simulink model "Final_year_project_mechanical_fault"  (R2024b)
settings: Solver=ode45  StartTime=0.0  StopTime=20  MaxStep=1e-4  RelTol=1e-3  EnableMultiTasking=on
libraries: spsACVoltageSourceLib x1, spsCurrentMeasurementLib x1, spsRMSLib x1, spsSinglePhaseAsynchronousMachineLib x1, spsVoltageMeasurementLib x1, spspowerguiLib x1
settings Model: Creator=Misty Porcupine  LastModifiedBy=Misty Porcupine
settings SolverCC: AlgebraicLoopSolver=TrustRegion
settings DataIOCC: LimitDataPoints=on  SaveFormat=Array  ReturnWorkspaceOutputs=off
settings OptimizationCC: LifeSpan=inf
settings DebuggingCC: UnderspecifiedInitializationDetection=Classic  MergeDetectMultiDrivingBlocksExec=none  SolverPrmCheckMsg=warning  UnconnectedInputMsg=warning  UnconnectedOutputMsg=warning  UnconnectedLineMsg=warning  SFUnexpectedBacktrackingDiag=warning  SFNoUnconditionalDefaultTransitionDiag=warning  SFExecutionAtInitializationDiag=none  ArithmeticOperatorsInVariantConditions=warning
settings HardwareCC: ProdBitPerPointer=32  ProdBitPerSizeT=32  ProdBitPerPtrDiffT=32  ProdLargestAtomicFloat=None  ProdIntDivRoundTo=Undefined  ProdEndianess=Unspecified  ProdWordSize=32  ProdHWDeviceType=32-bit Generic
settings ModelReferenceCC: PropagateSignalLabelsOutOfModel=off
settings SFSimCC: SimUseLocalCustomCode=off  CustomCodeUndefinedFunction=UseInterfaceOnly
settings RTWCC: RTWUseLocalCustomCode=off  GPUComputeCapability=3.5
settings CodeAppCC: StateflowObjectComments=on
settings GRTTargetCC: TargetLangStandard=C89/C90 (ANSI)
settings ConfigComp: CovMetricSettings=dw  CovSaveCumulativeToWorkspaceVar=on  CovSaveSingleToWorkspaceVar=on  CovExternalEMLEnable=off
settings SimscapeCC: SimscapeNormalizeSystem=off

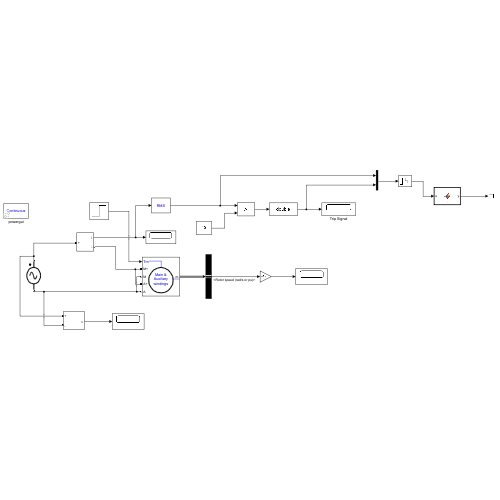
[thumbnail: Simulink's stored preview of the top-level diagram]
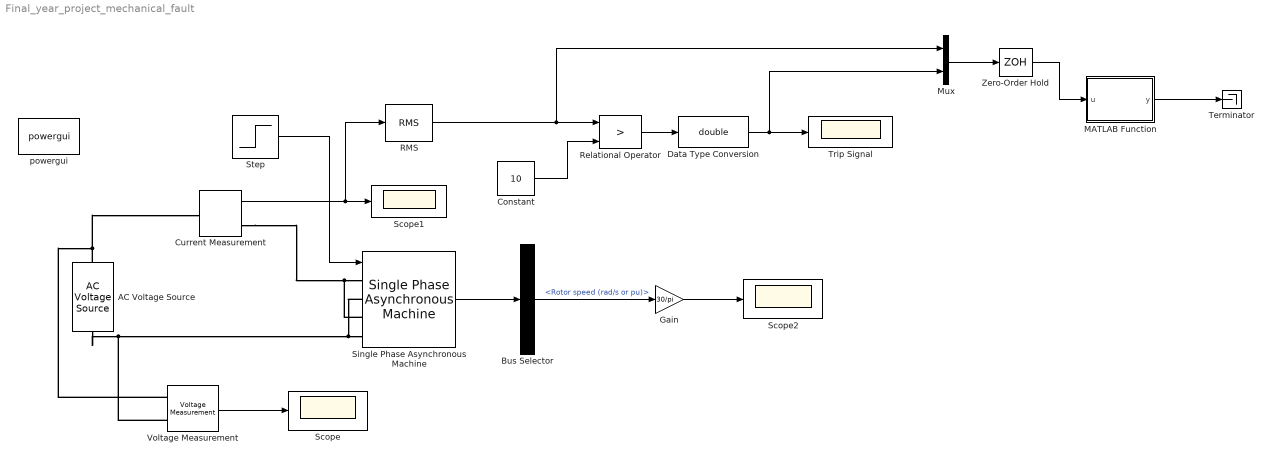
== system Final_year_project_mechanical_fault ==
  AC Voltage Source : spsACVoltageSourceLib/AC Voltage Source  Amplitude=100  Phase=0  Frequency=50  SampleTime=0  Measurements=None  BusType=swing  Pref=10e3  Qref=0  Qmin=-inf  Qmax=+inf
  Bus Selector : BusSelector  OutputSignals=Mechanical.Rotor speed (rad/s or pu)
  Constant : Constant  Value=10
  Current Measurement : spsCurrentMeasurementLib/Current Measurement  PhasorSimulation=off  OutputType=Complex  PSBequivalent=0
  Data Type Conversion : DataTypeConversion  OutDataTypeStr=double  SaturateOnIntegerOverflow=off  RndMeth=Floor
  Gain : Gain  Gain=30/pi
  MATLAB Function : MATLAB Function  TreatAsAtomicUnit=on
  Mux : Mux  Inputs=2
  RMS : spsRMSLib/RMS  TrueRMS=on  Freq=50  RMSInit=120  Ts=0
  Relational Operator : RelationalOperator  Operator=>  OutDataTypeStr=boolean  InputSameDT=off
  Scope : Scope
  Scope1 : Scope
  Scope2 : Scope
  Single Phase Asynchronous Machine : spsSinglePhaseAsynchronousMachineLib/Single Phase Asynchronous Machine  MechanicalLoad=Torque Tm  UNITS=SI  MachineType=Main & auxiliary windings  MeasurementBus=off  NominalParameters="[ .25*746  110  50]"  MainWindingStator="[2.02  7.4e-3]"  MainWindingRotor="[4.12  5.6e-3]"  MutualInductance=0.1772  AuxiliaryWinding="[7.14  8.5e-3]"  Mechanical="[0.0146  0  2 1.18]"  CapacitorStart="[2  254.7e-6]"  CapacitorRun="[18  21.1e-6]"  DisconnectionSpeed=75  InitialSpeed=0  DataType=SI  TsPowergui=0  TsBlock=-1
      settings: LibrarySourceBlock=|
      | sps_lib/Electrical Machines/Single Phase
      | Asynchronous Machine
  Step : Step  Time=0.25  Before=1  After=10  SampleTime=0
  Terminator : Terminator
  Trip Signal : Scope
  Voltage Measurement : spsVoltageMeasurementLib/Voltage Measurement  PhasorSimulation=off  OutputType=Complex  PSBequivalent=0
  Zero-Order Hold : ZeroOrderHold  SampleTime=15
  powergui : spspowerguiLib/powergui  Priority=1  SimulationMode=Continuous  SampleTime=50e-6  frequency=60  Iterations=50  frequencyindice=50  Pbase=100e6  ErrMax=1e-4  UnitsV=kV  UnitsW=MW  buscounter=0  FunctionMessages=off  echomessages=off  EnableUseOfTLC=off  CurrentSourceSwitches=off  DisableSnubberDevices=off  DisableRonSwitches=off  DisableVfSwitches=off  DisplayEquations=off  AutomaticDiscreteSolvers=off  SolverType=Tustin  Interpol=off  ExternalGateDelay=off  methode=off  Ts=0  x0status=blocks  SPID=off  SwTol=0  HookPort=off  NonlinearTolerance=1e-4  nMaxIteration=100  ContinueOnMaxIteration=off  RestoreLinks=warning  ResistiveCurrentMeasurement=off  Frange=[0:2:500]  Ylog=off  Xlog=on  ShowGrid=off  save=off  variable=ZData  structure=0  ZoomFFT=off  StartTime=0.0  cycles=1  DisplayStyle=1  fundamental=60  FreqAxis=off  MaxFrequency=1000  frequencyindicesteady=1  RmsSteady=1  display=off
  wires:
  Current Measurement/1 -> RMS/1, Scope1/1
  Step/1 -> Single Phase Asynchronous Machine/1
  Voltage Measurement/1 -> Scope/1
  Single Phase Asynchronous Machine/1 -> Bus Selector/1
  Bus Selector/1 -> Gain/1  "<Rotor speed (rad/s or pu)>"
  RMS/1 -> Mux/1, Relational Operator/1
  Constant/1 -> Relational Operator/2
  Gain/1 -> Scope2/1
  Relational Operator/1 -> Data Type Conversion/1
  Data Type Conversion/1 -> Mux/2, Trip Signal/1
  Mux/1 -> Zero-Order Hold/1
  Zero-Order Hold/1 -> MATLAB Function/1(u)
  MATLAB Function/1(y) -> Terminator/1
  connections:
  Voltage Measurement/LConn1 -- Current Measurement/LConn1 -- AC Voltage Source/RConn1
  Current Measurement/RConn1 -- Single Phase Asynchronous Machine/LConn3 -- Single Phase Asynchronous Machine/LConn1
  AC Voltage Source/LConn1 -- Voltage Measurement/LConn2 -- Single Phase Asynchronous Machine/LConn2 -- Single Phase Asynchronous Machine/LConn4

== matlab function Final_year_project_mechanical_fault/MATLAB Function ==
  data: u input; y output
function y = fcn(u)
coder.extrinsic('sendToThingSpeak');
y = 0;
y = sendToThingSpeak(u);
